simulink model "EV_Powertrain_Safety_Architecture"  (R2026b)
settings: Solver=VariableStepAuto
model workspace (MAT data in the model file):
  CAN_Bus = Simulink.Bus
  CAN_Bus.PreserveElementDimensions = 0
  CAN_Bus.Elements_internal(1) = Simulink.BusElement
  CAN_Bus.Elements_internal(1).DimensionsMode = 'Fixed'
  CAN_Bus.Elements_internal(1).DocUnits = 'Nm'
  CAN_Bus.Elements_internal(1).Name = 'Torque'
  CAN_Bus.Elements_internal(1).DataType_internal = 'ValueType: Torque'
  CAN_Bus.Elements_internal(1).Complexity = 'real'
  CAN_Bus.Elements_internal(1).Dimensions = 1
  CAN_Bus.Elements_internal(2) = Simulink.BusElement
  CAN_Bus.Elements_internal(2).DimensionsMode = 'Fixed'
  CAN_Bus.Elements_internal(2).DocUnits = 'degC'
  CAN_Bus.Elements_internal(2).Name = 'Temp_degC'
  CAN_Bus.Elements_internal(2).DataType_internal = 'ValueType: Temp_degC'
  CAN_Bus.Elements_internal(2).Complexity = 'real'
  CAN_Bus.Elements_internal(2).Dimensions = 1
  CAN_Bus.Elements_internal(3) = Simulink.BusElement
  CAN_Bus.Elements_internal(3).DimensionsMode = 'Fixed'
  CAN_Bus.Elements_internal(3).Name = 'Flag_Bool'
  CAN_Bus.Elements_internal(3).DataType_internal = 'boolean'
  CAN_Bus.Elements_internal(3).Complexity = 'real'
  CAN_Bus.Elements_internal(3).Dimensions = 1
  CAN_Bus.DataScope = 'Auto'
  Current_A = Simulink.ValueType
  Current_A.Unit = 'A'
  Pedal_Pct = Simulink.ValueType
  Pedal_Pct.Unit = '%'
  Temp_degC = Simulink.ValueType
  Temp_degC.Unit = 'degC'
  Three_Phase_Voltage_V = Simulink.ValueType
  Three_Phase_Voltage_V.Unit = 'V'
  Torque = Simulink.ValueType
  Torque.Unit = 'Nm'
settings Model: Creator=gokde  LastModifiedBy=gokde

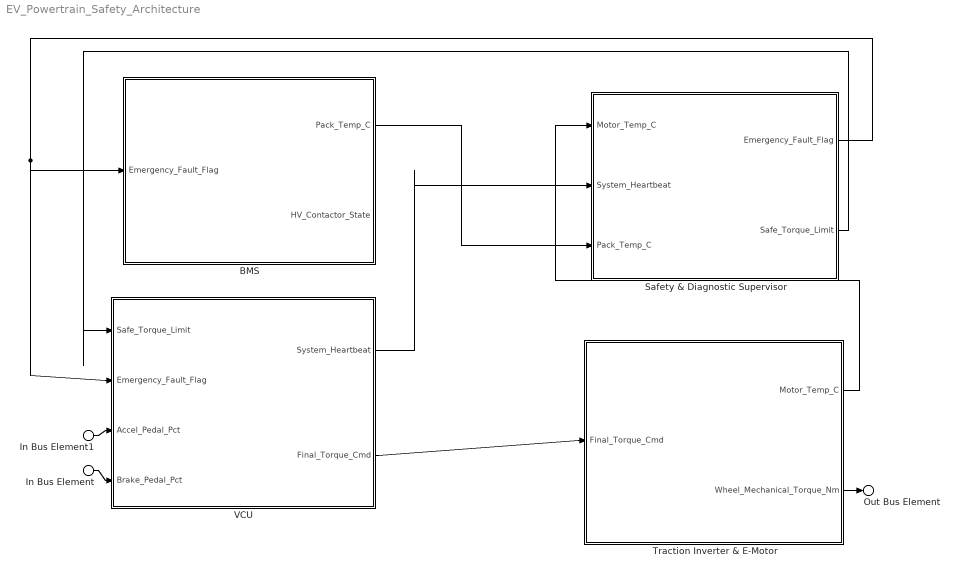
== system EV_Powertrain_Safety_Architecture ==
  In Bus Element1 : Inport  PortName=Accel_Pedal_Pct
  In Bus Element : Inport  Port=2  PortName=Brake_Pedal_Pct
  BMS : Subsystem
      settings: PortSchema="{\"entries\":[{\"content\":{\"headerSize\":26,\"margin\":15,\"minimumSpacing\":25,\"sides\":[{\"content\":{\"connectorIds\":[\"In1\"]},\"type\":\"ConnectorPlacement.EquallySpacedRectSide\",\"uuid\":\"b5e71f2c-f540-43cd-8ab9-859eadab86df\"},{\"content\":{\"connectorIds\":[\"Out1\",\"Out2\"],\"side\":\"RIGHT\"},\"type\":\"ConnectorPlacement.EquallySpacedRectSide\",\"uuid\":\"48767019-5cb7-46ef-9600-a821af9a3707\"},{\"content\":{\"side\":\"TOP\"},\"type\":\"ConnectorPlacement.EquallySpacedRectSide\",\"uuid\":\"e5d8e6fa-27bf-48d1-ab68-4adb692f8a92\"}]},\"type\":\"ConnectorPlacement.EquallySpacedConnector\",\"uuid\":\"f9a346ec-8fd8-4b98-9b35-247ccfc676b3\"}],\"packageUris\":[\"http://schema.mathworks.com/mf0/Connector/R2020b\"],\"version\":\"1.0\"}"
  Safety & Diagnostic Supervisor : Stateflow chart  TreatAsAtomicUnit=on
      settings: PortSchema="{\"entries\":[{\"content\":{\"headerSize\":26,\"margin\":15,\"minimumSpacing\":25,\"sides\":[{\"content\":{\"connectorIds\":[\"In1\",\"In2\",\"In3\"]},\"type\":\"ConnectorPlacement.EquallySpacedRectSide\",\"uuid\":\"b5e71f2c-f540-43cd-8ab9-859eadab86df\"},{\"content\":{\"connectorIds\":[\"Out1\",\"Out2\"],\"side\":\"RIGHT\"},\"type\":\"ConnectorPlacement.EquallySpacedRectSide\",\"uuid\":\"48767019-5cb7-46ef-9600-a821af9a3707\"},{\"content\":{\"side\":\"TOP\"},\"type\":\"ConnectorPlacement.EquallySpacedRectSide\",\"uuid\":\"e5d8e6fa-27bf-48d1-ab68-4adb692f8a92\"}]},\"type\":\"ConnectorPlacement.EquallySpacedConnector\",\"uuid\":\"f9a346ec-8fd8-4b98-9b35-247ccfc676b3\"}],\"packageUris\":[\"http://schema.mathworks.com/mf0/Connector/R2020b\"],\"version\":\"1.0\"}"
  Traction Inverter & E-Motor : Subsystem
      settings: PortSchema="{\"entries\":[{\"content\":{\"headerSize\":26,\"margin\":15,\"minimumSpacing\":25,\"sides\":[{\"content\":{\"connectorIds\":[\"In1\"]},\"type\":\"ConnectorPlacement.EquallySpacedRectSide\",\"uuid\":\"b5e71f2c-f540-43cd-8ab9-859eadab86df\"},{\"content\":{\"connectorIds\":[\"Out1\",\"Out2\"],\"side\":\"RIGHT\"},\"type\":\"ConnectorPlacement.EquallySpacedRectSide\",\"uuid\":\"48767019-5cb7-46ef-9600-a821af9a3707\"},{\"content\":{\"side\":\"TOP\"},\"type\":\"ConnectorPlacement.EquallySpacedRectSide\",\"uuid\":\"e5d8e6fa-27bf-48d1-ab68-4adb692f8a92\"}]},\"type\":\"ConnectorPlacement.EquallySpacedConnector\",\"uuid\":\"f9a346ec-8fd8-4b98-9b35-247ccfc676b3\"}],\"packageUris\":[\"http://schema.mathworks.com/mf0/Connector/R2020b\"],\"version\":\"1.0\"}"
  VCU : Subsystem
      settings: PortSchema="{\"entries\":[{\"content\":{\"headerSize\":26,\"margin\":15,\"minimumSpacing\":25,\"sides\":[{\"content\":{\"connectorIds\":[\"In1\",\"In2\",\"In3\",\"In4\"]},\"type\":\"ConnectorPlacement.EquallySpacedRectSide\",\"uuid\":\"b5e71f2c-f540-43cd-8ab9-859eadab86df\"},{\"content\":{\"connectorIds\":[\"Out1\",\"Out2\"],\"side\":\"RIGHT\"},\"type\":\"ConnectorPlacement.EquallySpacedRectSide\",\"uuid\":\"48767019-5cb7-46ef-9600-a821af9a3707\"},{\"content\":{\"side\":\"TOP\"},\"type\":\"ConnectorPlacement.EquallySpacedRectSide\",\"uuid\":\"e5d8e6fa-27bf-48d1-ab68-4adb692f8a92\"}]},\"type\":\"ConnectorPlacement.EquallySpacedConnector\",\"uuid\":\"f9a346ec-8fd8-4b98-9b35-247ccfc676b3\"}],\"packageUris\":[\"http://schema.mathworks.com/mf0/Connector/R2020b\"],\"version\":\"1.0\"}"
  Out Bus Element : Outport  PortName=Wheel_Mechanical_Torque_Nm
  wires:
  VCU/2(Final_Torque_Cmd) -> Traction Inverter & E-Motor/1(Final_Torque_Cmd)
  In Bus Element/1 -> VCU/4(Brake_Pedal_Pct)
  In Bus Element1/1 -> VCU/3(Accel_Pedal_Pct)
  Traction Inverter & E-Motor/2(Wheel_Mechanical_Torque_Nm) -> Out Bus Element/1
  Traction Inverter & E-Motor/1(Motor_Temp_C) -> Safety & Diagnostic Supervisor/1(Motor_Temp_C)
  BMS/1(Pack_Temp_C) -> Safety & Diagnostic Supervisor/3(Pack_Temp_C)
  VCU/1(System_Heartbeat) -> Safety & Diagnostic Supervisor/2(System_Heartbeat)
  Safety & Diagnostic Supervisor/1(Emergency_Fault_Flag) -> VCU/2(Emergency_Fault_Flag), BMS/1(Emergency_Fault_Flag)
  Safety & Diagnostic Supervisor/2(Safe_Torque_Limit) -> VCU/1(Safe_Torque_Limit)

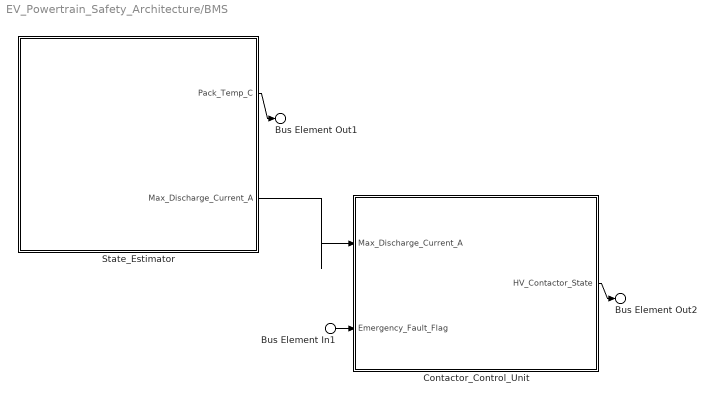
== system EV_Powertrain_Safety_Architecture/BMS ==
  Bus Element In1 : Inport  PortName=Emergency_Fault_Flag
  Contactor_Control_Unit : Subsystem
      settings: PortSchema="{\"entries\":[{\"content\":{\"headerSize\":26,\"margin\":15,\"minimumSpacing\":25,\"sides\":[{\"content\":{\"connectorIds\":[\"In1\",\"In2\"]},\"type\":\"ConnectorPlacement.EquallySpacedRectSide\",\"uuid\":\"b5e71f2c-f540-43cd-8ab9-859eadab86df\"},{\"content\":{\"connectorIds\":[\"Out1\"],\"side\":\"RIGHT\"},\"type\":\"ConnectorPlacement.EquallySpacedRectSide\",\"uuid\":\"48767019-5cb7-46ef-9600-a821af9a3707\"},{\"content\":{\"side\":\"TOP\"},\"type\":\"ConnectorPlacement.EquallySpacedRectSide\",\"uuid\":\"e5d8e6fa-27bf-48d1-ab68-4adb692f8a92\"}]},\"type\":\"ConnectorPlacement.EquallySpacedConnector\",\"uuid\":\"f9a346ec-8fd8-4b98-9b35-247ccfc676b3\"}],\"packageUris\":[\"http://schema.mathworks.com/mf0/Connector/R2020b\"],\"version\":\"1.0\"}"
  State_Estimator : Subsystem
      settings: PortSchema="{\"entries\":[{\"content\":{\"headerSize\":26,\"margin\":15,\"minimumSpacing\":25,\"sides\":[{\"content\":{},\"type\":\"ConnectorPlacement.EquallySpacedRectSide\",\"uuid\":\"b5e71f2c-f540-43cd-8ab9-859eadab86df\"},{\"content\":{\"connectorIds\":[\"Out2\",\"Out1\"],\"side\":\"RIGHT\"},\"type\":\"ConnectorPlacement.EquallySpacedRectSide\",\"uuid\":\"48767019-5cb7-46ef-9600-a821af9a3707\"},{\"content\":{\"side\":\"TOP\"},\"type\":\"ConnectorPlacement.EquallySpacedRectSide\",\"uuid\":\"e5d8e6fa-27bf-48d1-ab68-4adb692f8a92\"}]},\"type\":\"ConnectorPlacement.EquallySpacedConnector\",\"uuid\":\"f9a346ec-8fd8-4b98-9b35-247ccfc676b3\"}],\"packageUris\":[\"http://schema.mathworks.com/mf0/Connector/R2020b\"],\"version\":\"1.0\"}"
  Bus Element Out1 : Outport  PortName=Pack_Temp_C
  Bus Element Out2 : Outport  Port=2  PortName=HV_Contactor_State
  wires:
  State_Estimator/2(Pack_Temp_C) -> Bus Element Out1/1
  State_Estimator/1(Max_Discharge_Current_A) -> Contactor_Control_Unit/1(Max_Discharge_Current_A)
  Bus Element In1/1 -> Contactor_Control_Unit/2(Emergency_Fault_Flag)
  Contactor_Control_Unit/1(HV_Contactor_State) -> Bus Element Out2/1

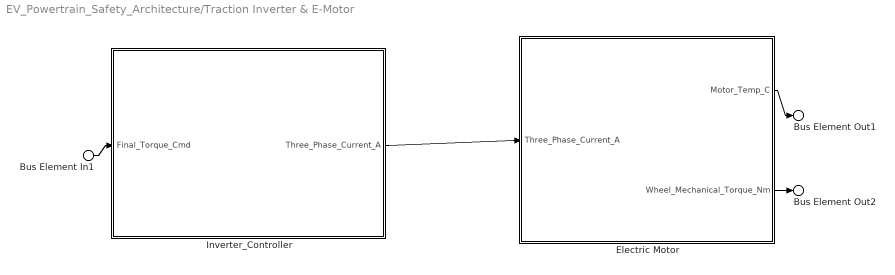
== system EV_Powertrain_Safety_Architecture/Traction Inverter & E-Motor ==
  Bus Element In1 : Inport  PortName=Final_Torque_Cmd
  Electric Motor : Subsystem
      settings: PortSchema="{\"entries\":[{\"content\":{\"headerSize\":26,\"margin\":15,\"minimumSpacing\":25,\"sides\":[{\"content\":{\"connectorIds\":[\"In1\"]},\"type\":\"ConnectorPlacement.EquallySpacedRectSide\",\"uuid\":\"b5e71f2c-f540-43cd-8ab9-859eadab86df\"},{\"content\":{\"connectorIds\":[\"Out1\",\"Out2\"],\"side\":\"RIGHT\"},\"type\":\"ConnectorPlacement.EquallySpacedRectSide\",\"uuid\":\"48767019-5cb7-46ef-9600-a821af9a3707\"},{\"content\":{\"side\":\"TOP\"},\"type\":\"ConnectorPlacement.EquallySpacedRectSide\",\"uuid\":\"e5d8e6fa-27bf-48d1-ab68-4adb692f8a92\"}]},\"type\":\"ConnectorPlacement.EquallySpacedConnector\",\"uuid\":\"f9a346ec-8fd8-4b98-9b35-247ccfc676b3\"}],\"packageUris\":[\"http://schema.mathworks.com/mf0/Connector/R2020b\"],\"version\":\"1.0\"}"
  Inverter_Controller : Subsystem
      settings: PortSchema="{\"entries\":[{\"content\":{\"headerSize\":26,\"margin\":15,\"minimumSpacing\":25,\"sides\":[{\"content\":{\"connectorIds\":[\"In1\"]},\"type\":\"ConnectorPlacement.EquallySpacedRectSide\",\"uuid\":\"b5e71f2c-f540-43cd-8ab9-859eadab86df\"},{\"content\":{\"connectorIds\":[\"Out1\"],\"side\":\"RIGHT\"},\"type\":\"ConnectorPlacement.EquallySpacedRectSide\",\"uuid\":\"48767019-5cb7-46ef-9600-a821af9a3707\"},{\"content\":{\"side\":\"TOP\"},\"type\":\"ConnectorPlacement.EquallySpacedRectSide\",\"uuid\":\"e5d8e6fa-27bf-48d1-ab68-4adb692f8a92\"}]},\"type\":\"ConnectorPlacement.EquallySpacedConnector\",\"uuid\":\"f9a346ec-8fd8-4b98-9b35-247ccfc676b3\"}],\"packageUris\":[\"http://schema.mathworks.com/mf0/Connector/R2020b\"],\"version\":\"1.0\"}"
  Bus Element Out1 : Outport  PortName=Motor_Temp_C
  Bus Element Out2 : Outport  Port=2  PortName=Wheel_Mechanical_Torque_Nm
  wires:
  Bus Element In1/1 -> Inverter_Controller/1(Final_Torque_Cmd)
  Inverter_Controller/1(Three_Phase_Current_A) -> Electric Motor/1(Three_Phase_Current_A)
  Electric Motor/1(Motor_Temp_C) -> Bus Element Out1/1
  Electric Motor/2(Wheel_Mechanical_Torque_Nm) -> Bus Element Out2/1

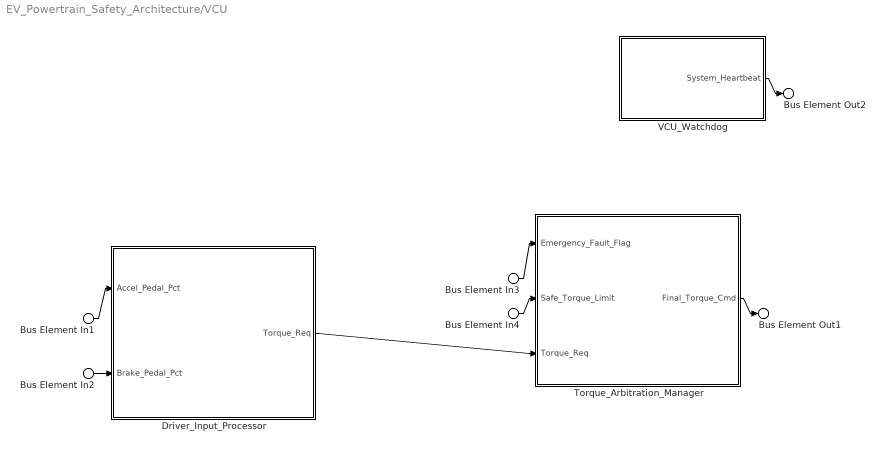
== system EV_Powertrain_Safety_Architecture/VCU ==
  Bus Element In4 : Inport  PortName=Safe_Torque_Limit
  Bus Element In3 : Inport  Port=2  PortName=Emergency_Fault_Flag
  Bus Element In1 : Inport  Port=3  PortName=Accel_Pedal_Pct
  Bus Element In2 : Inport  Port=4  PortName=Brake_Pedal_Pct
  Driver_Input_Processor : Subsystem
      settings: PortSchema="{\"entries\":[{\"content\":{\"headerSize\":26,\"margin\":15,\"minimumSpacing\":25,\"sides\":[{\"content\":{\"connectorIds\":[\"In1\",\"In2\"]},\"type\":\"ConnectorPlacement.EquallySpacedRectSide\",\"uuid\":\"b5e71f2c-f540-43cd-8ab9-859eadab86df\"},{\"content\":{\"connectorIds\":[\"Out1\"],\"side\":\"RIGHT\"},\"type\":\"ConnectorPlacement.EquallySpacedRectSide\",\"uuid\":\"48767019-5cb7-46ef-9600-a821af9a3707\"},{\"content\":{\"side\":\"TOP\"},\"type\":\"ConnectorPlacement.EquallySpacedRectSide\",\"uuid\":\"e5d8e6fa-27bf-48d1-ab68-4adb692f8a92\"}]},\"type\":\"ConnectorPlacement.EquallySpacedConnector\",\"uuid\":\"f9a346ec-8fd8-4b98-9b35-247ccfc676b3\"}],\"packageUris\":[\"http://schema.mathworks.com/mf0/Connector/R2020b\"],\"version\":\"1.0\"}"
  Torque_Arbitration_Manager : Subsystem
      settings: PortSchema="{\"entries\":[{\"content\":{\"headerSize\":26,\"margin\":15,\"minimumSpacing\":25,\"sides\":[{\"content\":{\"connectorIds\":[\"In1\",\"In2\",\"In3\"]},\"type\":\"ConnectorPlacement.EquallySpacedRectSide\",\"uuid\":\"b5e71f2c-f540-43cd-8ab9-859eadab86df\"},{\"content\":{\"connectorIds\":[\"Out1\"],\"side\":\"RIGHT\"},\"type\":\"ConnectorPlacement.EquallySpacedRectSide\",\"uuid\":\"48767019-5cb7-46ef-9600-a821af9a3707\"},{\"content\":{\"side\":\"TOP\"},\"type\":\"ConnectorPlacement.EquallySpacedRectSide\",\"uuid\":\"e5d8e6fa-27bf-48d1-ab68-4adb692f8a92\"}]},\"type\":\"ConnectorPlacement.EquallySpacedConnector\",\"uuid\":\"f9a346ec-8fd8-4b98-9b35-247ccfc676b3\"}],\"packageUris\":[\"http://schema.mathworks.com/mf0/Connector/R2020b\"],\"version\":\"1.0\"}"
  VCU_Watchdog : Subsystem
      settings: PortSchema="{\"entries\":[{\"content\":{\"headerSize\":26,\"margin\":15,\"minimumSpacing\":25,\"sides\":[{\"content\":{},\"type\":\"ConnectorPlacement.EquallySpacedRectSide\",\"uuid\":\"b5e71f2c-f540-43cd-8ab9-859eadab86df\"},{\"content\":{\"connectorIds\":[\"Out1\"],\"side\":\"RIGHT\"},\"type\":\"ConnectorPlacement.EquallySpacedRectSide\",\"uuid\":\"48767019-5cb7-46ef-9600-a821af9a3707\"},{\"content\":{\"side\":\"TOP\"},\"type\":\"ConnectorPlacement.EquallySpacedRectSide\",\"uuid\":\"e5d8e6fa-27bf-48d1-ab68-4adb692f8a92\"}]},\"type\":\"ConnectorPlacement.EquallySpacedConnector\",\"uuid\":\"f9a346ec-8fd8-4b98-9b35-247ccfc676b3\"}],\"packageUris\":[\"http://schema.mathworks.com/mf0/Connector/R2020b\"],\"version\":\"1.0\"}"
  Bus Element Out2 : Outport  PortName=System_Heartbeat
  Bus Element Out1 : Outport  Port=2  PortName=Final_Torque_Cmd
  wires:
  Driver_Input_Processor/1(Torque_Req) -> Torque_Arbitration_Manager/3(Torque_Req)
  Torque_Arbitration_Manager/1(Final_Torque_Cmd) -> Bus Element Out1/1
  Bus Element In1/1 -> Driver_Input_Processor/1(Accel_Pedal_Pct)
  Bus Element In2/1 -> Driver_Input_Processor/2(Brake_Pedal_Pct)
  Bus Element In4/1 -> Torque_Arbitration_Manager/2(Safe_Torque_Limit)
  Bus Element In3/1 -> Torque_Arbitration_Manager/1(Emergency_Fault_Flag)
  VCU_Watchdog/1(System_Heartbeat) -> Bus Element Out2/1

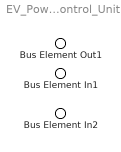
== system EV_Powertrain_Safety_Architecture/BMS/Contactor_Control_Unit ==
  Bus Element In1 : Inport  PortName=Max_Discharge_Current_A
  Bus Element In2 : Inport  Port=2  PortName=Emergency_Fault_Flag
  Bus Element Out1 : Outport  PortName=HV_Contactor_State

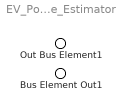
== system EV_Powertrain_Safety_Architecture/BMS/State_Estimator ==
  Bus Element Out1 : Outport  PortName=Max_Discharge_Current_A
  Out Bus Element1 : Outport  Port=2  PortName=Pack_Temp_C

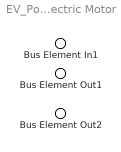
== system EV_Powertrain_Safety_Architecture/Traction Inverter & E-Motor/Electric Motor ==
  Bus Element In1 : Inport  PortName=Three_Phase_Current_A
  Bus Element Out1 : Outport  PortName=Motor_Temp_C
  Bus Element Out2 : Outport  Port=2  PortName=Wheel_Mechanical_Torque_Nm

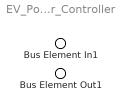
== system EV_Powertrain_Safety_Architecture/Traction Inverter & E-Motor/Inverter_Controller ==
  Bus Element In1 : Inport  PortName=Final_Torque_Cmd
  Bus Element Out1 : Outport  PortName=Three_Phase_Current_A

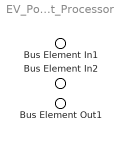
== system EV_Powertrain_Safety_Architecture/VCU/Driver_Input_Processor ==
  Bus Element In1 : Inport  PortName=Accel_Pedal_Pct
  Bus Element In2 : Inport  Port=2  PortName=Brake_Pedal_Pct
  Bus Element Out1 : Outport  PortName=Torque_Req

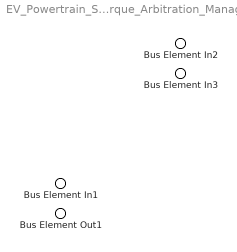
== system EV_Powertrain_Safety_Architecture/VCU/Torque_Arbitration_Manager ==
  Bus Element In3 : Inport  PortName=Emergency_Fault_Flag
  Bus Element In2 : Inport  Port=2  PortName=Safe_Torque_Limit
  Bus Element In1 : Inport  Port=3  PortName=Torque_Req
  Bus Element Out1 : Outport  PortName=Final_Torque_Cmd

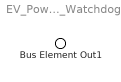
== system EV_Powertrain_Safety_Architecture/VCU/VCU_Watchdog ==
  Bus Element Out1 : Outport  PortName=System_Heartbeat

== stateflow chart EV_Powertrain_Safety_Architecture/Safety & Diagnostic Supervisor ==
  state NORMAL_DRIVE
    entry:
    Emergency_Fault_Flag = 0;
    Safe_Torque_Limit = 250;
  state THERMAL_DERATING
    entry:
    Emergency_Fault_Flag = 0;
    Safe_Torque_Limit = 100;
  state EMERGENCY_SAFE
    entry:
    Emergency_Fault_Flag = 1;
    Safe_Torque_Limit = 0;
  (default) -> NORMAL_DRIVE
  NORMAL_DRIVE -> THERMAL_DERATING [order 1] : [Motor_Temp_C > 90 || Pack_Temp_C > 50]
  THERMAL_DERATING -> NORMAL_DRIVE [order 1] : [Motor_Temp_C < 80 && Pack_Temp_C < 45]
  NORMAL_DRIVE -> EMERGENCY_SAFE [order 2] : [Motor_Temp_C > 120 || Pack_Temp_C > 65 || System_Heartbeat == 0]
  THERMAL_DERATING -> EMERGENCY_SAFE [order 2] : [System_Heartbeat == 0 || Motor_Temp_C > 120 || Pack_Temp_C > 65]
  data: Motor_Temp_C input Bus: CAN_Bus; System_Heartbeat input; Pack_Temp_C input Bus: CAN_Bus; Emergency_Fault_Flag output Bus: CAN_Bus; Safe_Torque_Limit output Bus: CAN_Bus
